simulink model "lfc_2area_pretty"  (R2026b)
settings: Solver=ode4  StopTime=p.Tend  FixedStep=p.dt
undefined symbols (not defined in the file): p
libraries: slpidlib x2
settings Model: Creator=arunkumar  LastModifiedBy=arunkumar

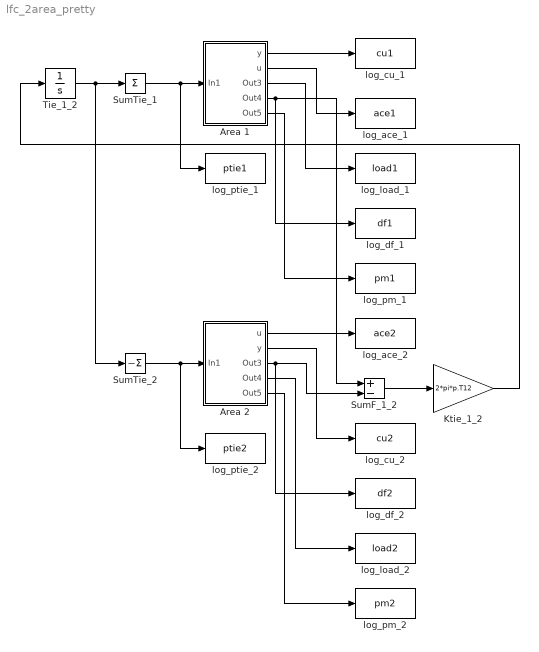
== system lfc_2area_pretty ==
  Area 1 : Subsystem
  Area 2 : Subsystem
  Ktie_1_2 : Gain  Gain=2*pi*p.T12
  SumF_1_2 : Sum  Inputs=+-
  SumTie_1 : Sum  Inputs=+
  SumTie_2 : Sum  Inputs=-
  Tie_1_2 : Integrator
  log_ace_1 : ToWorkspace  VariableName=ace1  SampleTime=-1
  log_ace_2 : ToWorkspace  VariableName=ace2  SampleTime=-1
  log_cu_1 : ToWorkspace  VariableName=cu1  SampleTime=-1
  log_cu_2 : ToWorkspace  VariableName=cu2  SampleTime=-1
  log_df_1 : ToWorkspace  VariableName=df1  SampleTime=-1
  log_df_2 : ToWorkspace  VariableName=df2  SampleTime=-1
  log_load_1 : ToWorkspace  VariableName=load1  SampleTime=-1
  log_load_2 : ToWorkspace  VariableName=load2  SampleTime=-1
  log_pm_1 : ToWorkspace  VariableName=pm1  SampleTime=-1
  log_pm_2 : ToWorkspace  VariableName=pm2  SampleTime=-1
  log_ptie_1 : ToWorkspace  VariableName=ptie1  SampleTime=-1
  log_ptie_2 : ToWorkspace  VariableName=ptie2  SampleTime=-1
  wires:
  SumF_1_2/1 -> Ktie_1_2/1
  Ktie_1_2/1 -> Tie_1_2/1
  Area 2/4(Out4) -> log_load_2/1
  Area 2/3(Out3) -> SumF_1_2/2, log_df_2/1
  Area 1/1(y) -> log_cu_1/1
  Area 2/1(u) -> log_ace_2/1
  Area 2/5(Out5) -> log_pm_2/1
  SumTie_2/1 -> Area 2/1(In1), log_ptie_2/1
  Area 1/5(Out5) -> log_pm_1/1
  Area 2/2(y) -> log_cu_2/1
  Area 1/4(Out4) -> SumF_1_2/1, log_df_1/1
  Area 1/3(Out3) -> log_load_1/1
  Tie_1_2/1 -> SumTie_1/1, SumTie_2/1
  Area 1/2(u) -> log_ace_1/1
  SumTie_1/1 -> Area 1/1(In1), log_ptie_1/1

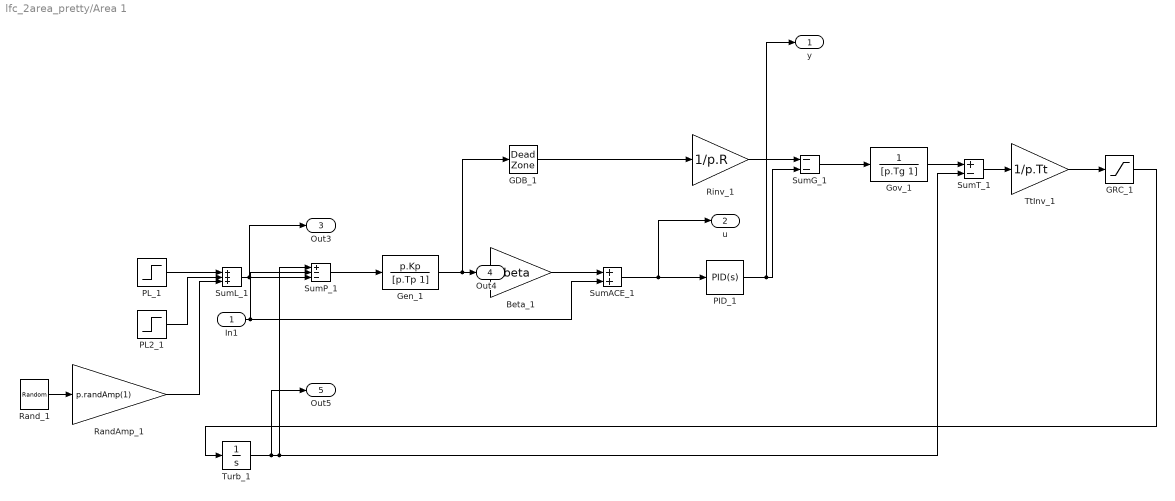
== system lfc_2area_pretty/Area 1 ==
  In1 : Inport
  Beta_1 : Gain  Gain=p.beta
  GDB_1 : DeadZone  LowerValue=-p.db  UpperValue=p.db
  GRC_1 : Saturate  UpperLimit=p.grc  LowerLimit=-p.grc
  Gen_1 : TransferFcn  Numerator=p.Kp  Denominator=[p.Tp 1]
  Gov_1 : TransferFcn  Numerator=1  Denominator=[p.Tg 1]
  PID_1 : slpidlib/PID Controller  Controller=PID  Form=Parallel  TimeDomain=Continuous-time  UseExternalTs=off  SampleTime=-1  IntegratorMethod=Forward Euler  FilterMethod=Forward Euler  ControllerParametersSource=internal  P=p.K(1,1)  I=p.K(1,2)  UseKiTs=off  D=p.K(1,3)  UseExternalDerivativeSource=off  N=p.N  UseFilter=on  TunerSelectOption=Transfer Function Based (PID Tuner App)  InitialConditionSource=internal  InitialConditionForIntegrator=0  InitialConditionForFilter=0  DifferentiatorICPrevScaledInput=0  ExternalReset=none  TrackingMode=off  Kt=1  LimitOutput=off  SatLimitsSource=internal  UpperSaturationLimit=inf  LowerSaturationLimit=-inf  LinearizeAsGain=on  AntiWindupMode=none  Kb=1  LimitIntegrator=off  UpperIntegratorSaturationLimit=inf  LowerIntegratorSaturationLimit=-inf  POutMin=[]  POutMax=[]  IOutMin=[]  IOutMax=[]  DOutMin=[]  DOutMax=[]  NOutMin=[]  NOutMax=[]  SumOutMin=[]  SumOutMax=[]  SaturationOutMin=[]  SaturationOutMax=[]  PParamMin=[]  PParamMax=[]  IParamMin=[]  IParamMax=[]  DParamMin=[]  DParamMax=[]  NParamMin=[]  NParamMax=[]  KbParamMin=[]  KbParamMax=[]  KtParamMin=[]  KtParamMax=[]  KbOutMin=[]  KbOutMax=[]  KtOutMin=[]  KtOutMax=[]  IntegratorOutMin=[]  IntegratorOutMax=[]  FilterOutMin=[]  FilterOutMax=[]  SumI1OutMin=[]  SumI1OutMax=[]  SumI2OutMin=[]  SumI2OutMax=[]  SumI3OutMin=[]  SumI3OutMax=[]  SumI4OutMin=[]  SumI4OutMax=[]  SumDOutMin=[]  SumDOutMax=[]  DifferentiatorOutMin=[]  DifferentiatorOutMax=[]  FilterDiffOutCoefMin=[]  FilterDiffOutCoefMax=[]  ReciprocalOutMin=[]  ReciprocalOutMax=[]  SumDenOutMin=[]  SumDenOutMax=[]  SumNumOutMin=[]  SumNumOutMax=[]  DivideOutMin=[]  DivideOutMax=[]  UdiffTsProdOutMin=[]  UdiffTsProdOutMax=[]  NTsProdOutMin=[]  NTsProdOutMax=[]  UintegralTsProdOutMin=[]  UintegralTsProdOutMax=[]  UngainTsProdOutMin=[]  UngainTsProdOutMax=[]  ClampingZeroOutDataTypeStr=Inherit: Inherit via back propagation  ClampingZeroOutMin=[]  ClampingZeroOutMax=[]  FilterDenConstantOutDataTypeStr=Inherit: Inherit via back propagation  FilterDenConstantOutMin=[]  FilterDenConstantOutMax=[]  PCopyOutDataTypeStr=Inherit: Inherit via back propagation  PCopyOutMin=[]  PCopyOutMax=[]  NCopyOutDataTypeStr=Inherit: Inherit via back propagation  NCopyOutMin=[]  NCopyOutMax=[]  IntegratorContinuousStateAttributes=''  IntegratorStateMustResolveToSignalObject=off  IntegratorRTWStateStorageClass=Auto  FilterContinuousStateAttributes=''  FilterStateMustResolveToSignalObject=off  FilterRTWStateStorageClass=Auto  ParallelPVariant=InternalParameters  IdealPVariant=Disabled  IVariant=InternalParameters  DVariant=InternalParameters  IntegratorVariant=Continuous  SatVariant=Disabled  AWVariant=Passthrough  PCopyVariant=Disabled  TRVariant=Disabled  FdbkBlocksVariant=Forward  IdealPFdbkVariant=Disabled  SatFdbkVariant=Disabled  DerivativeFilterVariant=ContFilter  NVariant=InternalParameters  NCopyVariant=Disabled  FilterICVariant=InternalICsFilter  IntegratorICVariant=InternalICs  ExternalResetVariant=Disabled  TRSumVariant=Passthrough  SumFdbkVariant=Disabled  SumVariant=Sum_PID  TsampFilterVariant=InternalTs  TsampNgainVariant=Passthrough  TsampIntegralVariant=Disabled_SignalSpec  ExternalSaturationOutDataTypeStr=Inherit: Same as second input  DerivativeSourceVariant=ErrorSignal  PreIntVariant=InternalPreInt
  PL2_1 : Step  Time=p.tL2  FinalValue=p.dPL2(1)  SampleTime=0
  PL_1 : Step  Time=0  FinalValue=p.dPL(1)  SampleTime=0
  RandAmp_1 : Gain  Gain=p.randAmp(1)
  Rand_1 : UniformRandomNumber  Seed=p.randSeed+1  SampleTime=p.randTs
  Rinv_1 : Gain  Gain=1/p.R
  SumACE_1 : Sum
  SumG_1 : Sum  Inputs=--
  SumL_1 : Sum  Inputs=+++
  SumP_1 : Sum  Inputs=+--
  SumT_1 : Sum  Inputs=+-
  TtInv_1 : Gain  Gain=1/p.Tt
  Turb_1 : Integrator
  y : Outport
  u : Outport  Port=2
  Out3 : Outport  Port=3
  Out4 : Outport  Port=4
  Out5 : Outport  Port=5
  wires:
  RandAmp_1/1 -> SumL_1/3
  Rinv_1/1 -> SumG_1/1
  PL2_1/1 -> SumL_1/2
  SumACE_1/1 -> u/1, PID_1/1
  GDB_1/1 -> Rinv_1/1
  SumP_1/1 -> Gen_1/1
  PID_1/1 -> y/1, SumG_1/2
  GRC_1/1 -> Turb_1/1
  Turb_1/1 -> Out5/1, SumP_1/1, SumT_1/2
  SumT_1/1 -> TtInv_1/1
  PL_1/1 -> SumL_1/1
  In1/1 -> SumACE_1/2, SumP_1/2
  Beta_1/1 -> SumACE_1/1
  Gen_1/1 -> GDB_1/1, Beta_1/1, Out4/1
  Gov_1/1 -> SumT_1/1
  SumL_1/1 -> Out3/1, SumP_1/3
  Rand_1/1 -> RandAmp_1/1
  TtInv_1/1 -> GRC_1/1
  SumG_1/1 -> Gov_1/1

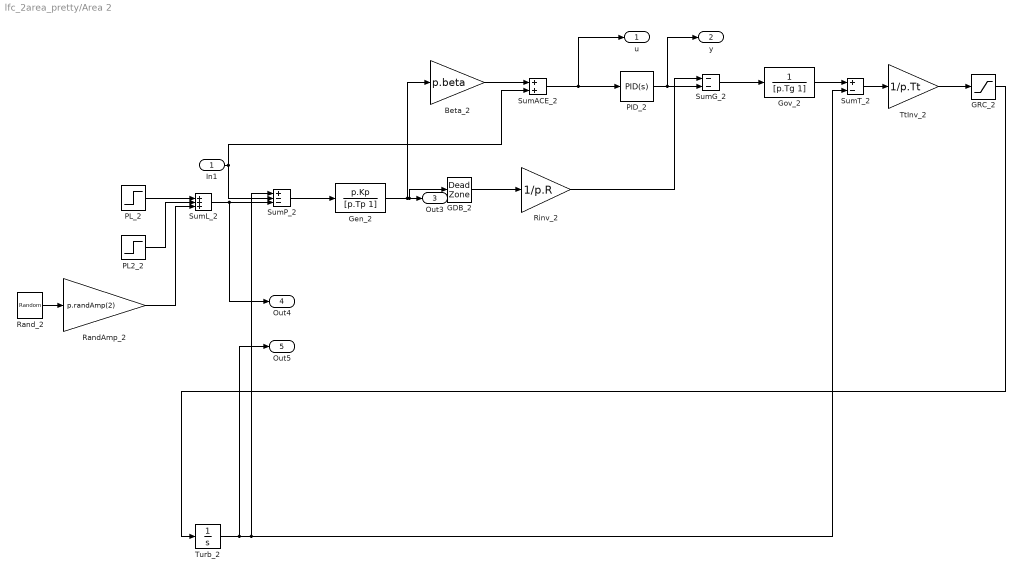
== system lfc_2area_pretty/Area 2 ==
  In1 : Inport
  Beta_2 : Gain  Gain=p.beta
  GDB_2 : DeadZone  LowerValue=-p.db  UpperValue=p.db
  GRC_2 : Saturate  UpperLimit=p.grc  LowerLimit=-p.grc
  Gen_2 : TransferFcn  Numerator=p.Kp  Denominator=[p.Tp 1]
  Gov_2 : TransferFcn  Numerator=1  Denominator=[p.Tg 1]
  PID_2 : slpidlib/PID Controller  Controller=PID  Form=Parallel  TimeDomain=Continuous-time  UseExternalTs=off  SampleTime=-1  IntegratorMethod=Forward Euler  FilterMethod=Forward Euler  ControllerParametersSource=internal  P=p.K(2,1)  I=p.K(2,2)  UseKiTs=off  D=p.K(2,3)  UseExternalDerivativeSource=off  N=p.N  UseFilter=on  TunerSelectOption=Transfer Function Based (PID Tuner App)  InitialConditionSource=internal  InitialConditionForIntegrator=0  InitialConditionForFilter=0  DifferentiatorICPrevScaledInput=0  ExternalReset=none  TrackingMode=off  Kt=1  LimitOutput=off  SatLimitsSource=internal  UpperSaturationLimit=inf  LowerSaturationLimit=-inf  LinearizeAsGain=on  AntiWindupMode=none  Kb=1  LimitIntegrator=off  UpperIntegratorSaturationLimit=inf  LowerIntegratorSaturationLimit=-inf  POutMin=[]  POutMax=[]  IOutMin=[]  IOutMax=[]  DOutMin=[]  DOutMax=[]  NOutMin=[]  NOutMax=[]  SumOutMin=[]  SumOutMax=[]  SaturationOutMin=[]  SaturationOutMax=[]  PParamMin=[]  PParamMax=[]  IParamMin=[]  IParamMax=[]  DParamMin=[]  DParamMax=[]  NParamMin=[]  NParamMax=[]  KbParamMin=[]  KbParamMax=[]  KtParamMin=[]  KtParamMax=[]  KbOutMin=[]  KbOutMax=[]  KtOutMin=[]  KtOutMax=[]  IntegratorOutMin=[]  IntegratorOutMax=[]  FilterOutMin=[]  FilterOutMax=[]  SumI1OutMin=[]  SumI1OutMax=[]  SumI2OutMin=[]  SumI2OutMax=[]  SumI3OutMin=[]  SumI3OutMax=[]  SumI4OutMin=[]  SumI4OutMax=[]  SumDOutMin=[]  SumDOutMax=[]  DifferentiatorOutMin=[]  DifferentiatorOutMax=[]  FilterDiffOutCoefMin=[]  FilterDiffOutCoefMax=[]  ReciprocalOutMin=[]  ReciprocalOutMax=[]  SumDenOutMin=[]  SumDenOutMax=[]  SumNumOutMin=[]  SumNumOutMax=[]  DivideOutMin=[]  DivideOutMax=[]  UdiffTsProdOutMin=[]  UdiffTsProdOutMax=[]  NTsProdOutMin=[]  NTsProdOutMax=[]  UintegralTsProdOutMin=[]  UintegralTsProdOutMax=[]  UngainTsProdOutMin=[]  UngainTsProdOutMax=[]  ClampingZeroOutDataTypeStr=Inherit: Inherit via back propagation  ClampingZeroOutMin=[]  ClampingZeroOutMax=[]  FilterDenConstantOutDataTypeStr=Inherit: Inherit via back propagation  FilterDenConstantOutMin=[]  FilterDenConstantOutMax=[]  PCopyOutDataTypeStr=Inherit: Inherit via back propagation  PCopyOutMin=[]  PCopyOutMax=[]  NCopyOutDataTypeStr=Inherit: Inherit via back propagation  NCopyOutMin=[]  NCopyOutMax=[]  IntegratorContinuousStateAttributes=''  IntegratorStateMustResolveToSignalObject=off  IntegratorRTWStateStorageClass=Auto  FilterContinuousStateAttributes=''  FilterStateMustResolveToSignalObject=off  FilterRTWStateStorageClass=Auto  ParallelPVariant=InternalParameters  IdealPVariant=Disabled  IVariant=InternalParameters  DVariant=InternalParameters  IntegratorVariant=Continuous  SatVariant=Disabled  AWVariant=Passthrough  PCopyVariant=Disabled  TRVariant=Disabled  FdbkBlocksVariant=Forward  IdealPFdbkVariant=Disabled  SatFdbkVariant=Disabled  DerivativeFilterVariant=ContFilter  NVariant=InternalParameters  NCopyVariant=Disabled  FilterICVariant=InternalICsFilter  IntegratorICVariant=InternalICs  ExternalResetVariant=Disabled  TRSumVariant=Passthrough  SumFdbkVariant=Disabled  SumVariant=Sum_PID  TsampFilterVariant=InternalTs  TsampNgainVariant=Passthrough  TsampIntegralVariant=Disabled_SignalSpec  ExternalSaturationOutDataTypeStr=Inherit: Same as second input  DerivativeSourceVariant=ErrorSignal  PreIntVariant=InternalPreInt
  PL2_2 : Step  Time=p.tL2  FinalValue=p.dPL2(2)  SampleTime=0
  PL_2 : Step  Time=0  FinalValue=p.dPL(2)  SampleTime=0
  RandAmp_2 : Gain  Gain=p.randAmp(2)
  Rand_2 : UniformRandomNumber  Seed=p.randSeed+2  SampleTime=p.randTs
  Rinv_2 : Gain  Gain=1/p.R
  SumACE_2 : Sum
  SumG_2 : Sum  Inputs=--
  SumL_2 : Sum  Inputs=+++
  SumP_2 : Sum  Inputs=+--
  SumT_2 : Sum  Inputs=+-
  TtInv_2 : Gain  Gain=1/p.Tt
  Turb_2 : Integrator
  u : Outport
  y : Outport  Port=2
  Out3 : Outport  Port=3
  Out4 : Outport  Port=4
  Out5 : Outport  Port=5
  wires:
  PL2_2/1 -> SumL_2/2
  SumP_2/1 -> Gen_2/1
  PL_2/1 -> SumL_2/1
  Rinv_2/1 -> SumG_2/1
  SumG_2/1 -> Gov_2/1
  GDB_2/1 -> Rinv_2/1
  GRC_2/1 -> Turb_2/1
  Rand_2/1 -> RandAmp_2/1
  RandAmp_2/1 -> SumL_2/3
  SumL_2/1 -> Out4/1, SumP_2/3
  PID_2/1 -> y/1, SumG_2/2
  TtInv_2/1 -> GRC_2/1
  Gen_2/1 -> GDB_2/1, Out3/1, Beta_2/1
  SumACE_2/1 -> u/1, PID_2/1
  Turb_2/1 -> Out5/1, SumP_2/1, SumT_2/2
  Beta_2/1 -> SumACE_2/1
  Gov_2/1 -> SumT_2/1
  In1/1 -> SumACE_2/2, SumP_2/2
  SumT_2/1 -> TtInv_2/1
